simulink model "SNS_WinnerSlice_R8"  (R2025a)
settings: Solver=ode1  StartTime=0.0  StopTime=22  FixedStep=0.002  RelTol=1e-3
libraries: SNS_Library_R2025a x106, simulink x6
(part 1 of 2)
Description:
  | Reduced winner slice: round8_best3.json human circuit in the redesigned SNS_Library architecture. See reports_20261016/sns_simulink/.
settings Model: Creator=ben bolen  LastModifiedBy=ben bolen

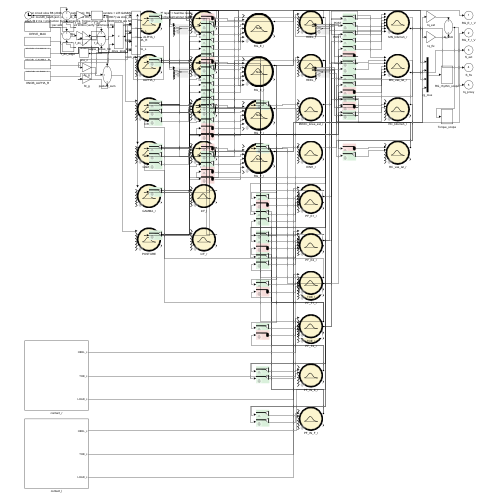
[thumbnail: Simulink's stored preview of the top-level diagram]
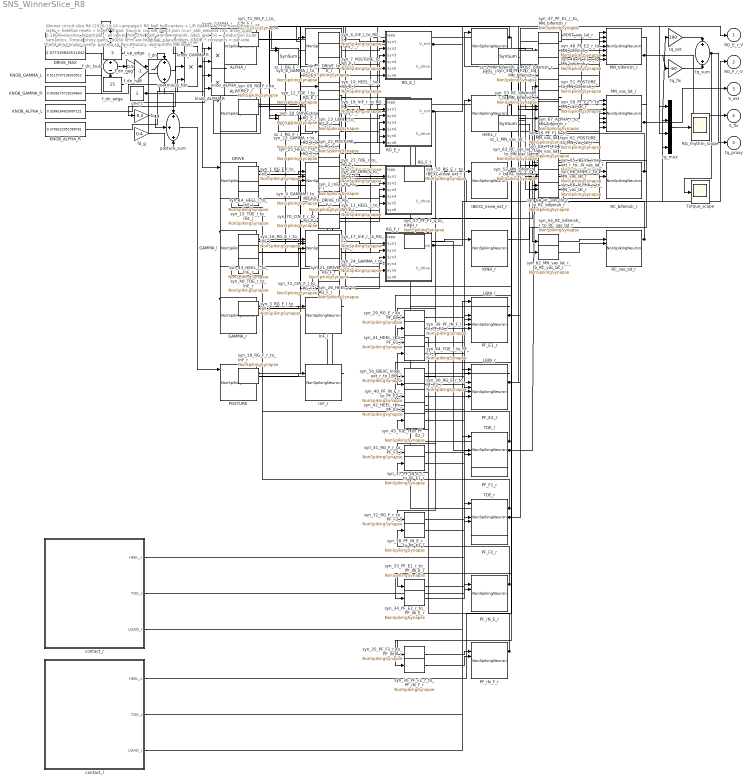
== system SNS_WinnerSlice_R8 ==
  note: Winner circuit slice R8 (2026-10-16 campaign): RG NaP half-centers + L/R GAMMA/ALPHA hand drive + PF layer + heel/toe resets + knee MN pair.
      | Source: round8_best3.json (curr_s8b_wean04 t35, drive_scale 0.3807) via slice_export.json - all values from the built winner network.
      | ode1 @ 2 ms = production Euler semantics. Torque proxy gains 190/60 N*m are NOMINAL placeholders.
      | KNOB_* constants = per-side hand-drive knobs (verify: gamma x4 flips RG duty; alpha shifts MN level).
  ALPHA_l : SNS_Library_R2025a/NonSpikingNeuron  Vrest=0  Gm=1  Cm=100  Thr=0  Slope=5
  ALPHA_r : SNS_Library_R2025a/NonSpikingNeuron  Vrest=0  Gm=1  Cm=100  Thr=0  Slope=5
  CIN_F_l : SNS_Library_R2025a/NonSpikingNeuron  Vrest=0  Gm=1  Cm=50  Thr=0  Slope=5
  CIN_F_r : SNS_Library_R2025a/NonSpikingNeuron  Vrest=0  Gm=1  Cm=50  Thr=0  Slope=5
  DRIVE : SNS_Library_R2025a/NonSpikingNeuron  Vrest=0  Gm=1  Cm=100  Thr=0  Slope=5
  DRIVE_MAX : Constant  Value=2.077319843511042
  GAMMA_l : SNS_Library_R2025a/NonSpikingNeuron  Vrest=0  Gm=1  Cm=100  Thr=0  Slope=5
  GAMMA_r : SNS_Library_R2025a/NonSpikingNeuron  Vrest=0  Gm=1  Cm=100  Thr=0  Slope=5
  HEEL_l : SNS_Library_R2025a/NonSpikingNeuron  Vrest=0  Gm=1  Cm=40  Thr=0  Slope=5
  HEEL_r : SNS_Library_R2025a/NonSpikingNeuron  Vrest=0  Gm=1  Cm=40  Thr=0  Slope=5
  IBEXC_knee_ext_r : SNS_Library_R2025a/NonSpikingNeuron  Vrest=0  Gm=1  Cm=50  Thr=0  Slope=5
  InE_l : SNS_Library_R2025a/NonSpikingNeuron  Vrest=0  Gm=1  Cm=50  Thr=0  Slope=5
  InE_r : SNS_Library_R2025a/NonSpikingNeuron  Vrest=0  Gm=1  Cm=50  Thr=0  Slope=5
  InF_l : SNS_Library_R2025a/NonSpikingNeuron  Vrest=0  Gm=1  Cm=50  Thr=0  Slope=5
  InF_r : SNS_Library_R2025a/NonSpikingNeuron  Vrest=0  Gm=1  Cm=50  Thr=0  Slope=5
  KINH_r : SNS_Library_R2025a/NonSpikingNeuron  Vrest=0  Gm=1  Cm=50  Thr=0  Slope=5
  KNOB_ALPHA_L : Constant  Value=0.3286184629397121
  KNOB_ALPHA_R : Constant  Value=0.3706222051599761
  KNOB_GAMMA_L : Constant  Value=0.5115737136333512
  KNOB_GAMMA_R : Constant  Value=0.3036175720234663
  LBIN_l : SNS_Library_R2025a/NonSpikingNeuron  Vrest=0  Gm=1  Cm=50  Thr=0  Slope=5
  LBIN_r : SNS_Library_R2025a/NonSpikingNeuron  Vrest=0  Gm=1  Cm=50  Thr=0  Slope=5
  MN_bifemsh_r : SNS_Library_R2025a/NonSpikingNeuron  Vrest=0  Gm=1  Cm=30  Thr=0  Slope=5
  MN_vas_lat_r : SNS_Library_R2025a/NonSpikingNeuron  Vrest=0  Gm=1  Cm=30  Thr=0  Slope=5
  PF_E1_r : SNS_Library_R2025a/NonSpikingNeuron  Vrest=0  Gm=1  Cm=48  Thr=0  Slope=5
  PF_E2_r : SNS_Library_R2025a/NonSpikingNeuron  Vrest=0  Gm=1  Cm=72  Thr=0  Slope=5
  PF_F1_r : SNS_Library_R2025a/NonSpikingNeuron  Vrest=0  Gm=1  Cm=72  Thr=0  Slope=5
  PF_F2_r : SNS_Library_R2025a/NonSpikingNeuron  Vrest=0  Gm=1  Cm=128  Thr=0  Slope=5
  PF_IN_E_r : SNS_Library_R2025a/NonSpikingNeuron  Vrest=0  Gm=1  Cm=80  Thr=0  Slope=5
  PF_IN_F_r : SNS_Library_R2025a/NonSpikingNeuron  Vrest=0  Gm=1  Cm=80  Thr=0  Slope=5
  POSTURE : SNS_Library_R2025a/NonSpikingNeuron  Vrest=0  Gm=1  Cm=100  Thr=0  Slope=5
  POST_bifemsh_r : Constant  Value=0
  POST_vas_lat_r : Constant  Value=0
  RC_bifemsh_r : SNS_Library_R2025a/NonSpikingNeuron  Vrest=0  Gm=1  Cm=30  Thr=0  Slope=5
  RC_vas_lat_r : SNS_Library_R2025a/NonSpikingNeuron  Vrest=0  Gm=1  Cm=30  Thr=0  Slope=5
  RG_E_l : Subsystem  mask(SNS NapNeuron (RG soma)){Vrest=0, Gm=1, Cm=50, Thr=0, Slope=5, gIon=12, eIon=8, kM=1, sM=0.8, eM=2, kH=1, sH=-2, eH=3.5, tauH=842.083318953, h0=0.000911051194401}
      mask prompts: Vrest "Resting potential Vrest (mV)"; Gm "Membrane conductance Gm (uS)"; Cm "Membrane capacitance Cm (nF)"; Thr "Saturation threshold Thr (mV)"; Slope "Saturation slope (1/mV)"; gIon "NaP conductance g_ion (uS)"; eIon "NaP reversal e_ion (mV)"; kM "m-gate k_m"; sM "m-gate slope_m (1/mV)"; eM "m-gate midpoint e_m (mV)"; kH "h-gate k_h"; sH "h-gate slope_h (1/mV)"; eH "h-gate midpoint e_h (mV)"; tauH "h-gate time constant tau_h (ms), FIXED"; h0 "initial h"
      mask help: Persistent-Na non-spiking neuron, fixed tau_h (sns_toolbox NonSpikingNeuronWithPersistentSodiumChannel under SNS_NumpyFixedTau = the production RG stepper). Same port conventions as SNS_Library/NonSpikingNeuron: Iapp [nA] + syn1..6, outputs V [mV] and S(V).
      mask Display:
      | t_ = linspace(0, 2*pi, 73);
      | patch(0.95*cos(t_), 0.95*sin(t_), [0 0 0]);
      | patch(0.84*cos(t_), 0.84*sin(t_), [0.99 0.96 0.81]);
      | x_ = linspace(-0.55, 0.55, 61);
      | y_ = -0.20 + 0.40*exp(-((x_+0.08)/0.26).^2);
      | color('black');
      | plot(x_, y_);
      | plot([-0.55 0.55], [-0.20 -0.20]);
      | disp('NaP');
  RG_E_r : Subsystem  mask(SNS NapNeuron (RG soma)){Vrest=0, Gm=1, Cm=50, Thr=0, Slope=5, gIon=12, eIon=8, kM=1, sM=0.8, eM=2, kH=1, sH=-2, eH=3.5, tauH=842.083318953, h0=0.000911051194401}
      mask prompts: Vrest "Resting potential Vrest (mV)"; Gm "Membrane conductance Gm (uS)"; Cm "Membrane capacitance Cm (nF)"; Thr "Saturation threshold Thr (mV)"; Slope "Saturation slope (1/mV)"; gIon "NaP conductance g_ion (uS)"; eIon "NaP reversal e_ion (mV)"; kM "m-gate k_m"; sM "m-gate slope_m (1/mV)"; eM "m-gate midpoint e_m (mV)"; kH "h-gate k_h"; sH "h-gate slope_h (1/mV)"; eH "h-gate midpoint e_h (mV)"; tauH "h-gate time constant tau_h (ms), FIXED"; h0 "initial h"
      mask help: Persistent-Na non-spiking neuron, fixed tau_h (sns_toolbox NonSpikingNeuronWithPersistentSodiumChannel under SNS_NumpyFixedTau = the production RG stepper). Same port conventions as SNS_Library/NonSpikingNeuron: Iapp [nA] + syn1..6, outputs V [mV] and S(V).
      mask Display:
      | t_ = linspace(0, 2*pi, 73);
      | patch(0.95*cos(t_), 0.95*sin(t_), [0 0 0]);
      | patch(0.84*cos(t_), 0.84*sin(t_), [0.99 0.96 0.81]);
      | x_ = linspace(-0.55, 0.55, 61);
      | y_ = -0.20 + 0.40*exp(-((x_+0.08)/0.26).^2);
      | color('black');
      | plot(x_, y_);
      | plot([-0.55 0.55], [-0.20 -0.20]);
      | disp('NaP');
  RG_F_l : Subsystem  mask(SNS NapNeuron (RG soma)){Vrest=0, Gm=1, Cm=50, Thr=0, Slope=5, gIon=12, eIon=8, kM=1, sM=0.8, eM=2, kH=1, sH=-2, eH=3.5, tauH=842.083318953, h0=0.000911051194401}
      mask prompts: Vrest "Resting potential Vrest (mV)"; Gm "Membrane conductance Gm (uS)"; Cm "Membrane capacitance Cm (nF)"; Thr "Saturation threshold Thr (mV)"; Slope "Saturation slope (1/mV)"; gIon "NaP conductance g_ion (uS)"; eIon "NaP reversal e_ion (mV)"; kM "m-gate k_m"; sM "m-gate slope_m (1/mV)"; eM "m-gate midpoint e_m (mV)"; kH "h-gate k_h"; sH "h-gate slope_h (1/mV)"; eH "h-gate midpoint e_h (mV)"; tauH "h-gate time constant tau_h (ms), FIXED"; h0 "initial h"
      mask help: Persistent-Na non-spiking neuron, fixed tau_h (sns_toolbox NonSpikingNeuronWithPersistentSodiumChannel under SNS_NumpyFixedTau = the production RG stepper). Same port conventions as SNS_Library/NonSpikingNeuron: Iapp [nA] + syn1..6, outputs V [mV] and S(V).
      mask Display:
      | t_ = linspace(0, 2*pi, 73);
      | patch(0.95*cos(t_), 0.95*sin(t_), [0 0 0]);
      | patch(0.84*cos(t_), 0.84*sin(t_), [0.99 0.96 0.81]);
      | x_ = linspace(-0.55, 0.55, 61);
      | y_ = -0.20 + 0.40*exp(-((x_+0.08)/0.26).^2);
      | color('black');
      | plot(x_, y_);
      | plot([-0.55 0.55], [-0.20 -0.20]);
      | disp('NaP');
  RG_F_r : Subsystem  mask(SNS NapNeuron (RG soma)){Vrest=0, Gm=1, Cm=50, Thr=0, Slope=5, gIon=12, eIon=8, kM=1, sM=0.8, eM=2, kH=1, sH=-2, eH=3.5, tauH=842.083318953, h0=0.000911051194401}
      mask prompts: Vrest "Resting potential Vrest (mV)"; Gm "Membrane conductance Gm (uS)"; Cm "Membrane capacitance Cm (nF)"; Thr "Saturation threshold Thr (mV)"; Slope "Saturation slope (1/mV)"; gIon "NaP conductance g_ion (uS)"; eIon "NaP reversal e_ion (mV)"; kM "m-gate k_m"; sM "m-gate slope_m (1/mV)"; eM "m-gate midpoint e_m (mV)"; kH "h-gate k_h"; sH "h-gate slope_h (1/mV)"; eH "h-gate midpoint e_h (mV)"; tauH "h-gate time constant tau_h (ms), FIXED"; h0 "initial h"
      mask help: Persistent-Na non-spiking neuron, fixed tau_h (sns_toolbox NonSpikingNeuronWithPersistentSodiumChannel under SNS_NumpyFixedTau = the production RG stepper). Same port conventions as SNS_Library/NonSpikingNeuron: Iapp [nA] + syn1..6, outputs V [mV] and S(V).
      mask Display:
      | t_ = linspace(0, 2*pi, 73);
      | patch(0.95*cos(t_), 0.95*sin(t_), [0 0 0]);
      | patch(0.84*cos(t_), 0.84*sin(t_), [0.99 0.96 0.81]);
      | x_ = linspace(-0.55, 0.55, 61);
      | y_ = -0.20 + 0.40*exp(-((x_+0.08)/0.26).^2);
      | color('black');
      | plot(x_, y_);
      | plot([-0.55 0.55], [-0.20 -0.20]);
      | disp('NaP');
  RG_rhythm_scope : Scope
  TOE_l : SNS_Library_R2025a/NonSpikingNeuron  Vrest=0  Gm=1  Cm=40  Thr=0  Slope=5
  TOE_r : SNS_Library_R2025a/NonSpikingNeuron  Vrest=0  Gm=1  Cm=40  Thr=0  Slope=5
  Torque_scope : Scope
  clock1 : Clock
  contact_l : Subsystem  Description=Foot-contact script (lag 0.50 cycle): stylized stance pattern, production cadence; runner-shaped port currents incl. contact_onset kicks.
  contact_r : Subsystem  Description=Foot-contact script (lag 0.00 cycle): stylized stance pattern, production cadence; runner-shaped port currents incl. contact_onset kicks.
  drive_prod : Product  Inputs=3
  f_dn : Saturate  UpperLimit=1  LowerLimit=0
  f_dn_edge : Constant  Value=15
  f_dn_half : Gain  Gain=0.5
  f_dn_neg : Gain  Gain=-1
  f_dn_tsub : Sum  Inputs=+-
  f_up : Saturate  UpperLimit=1  LowerLimit=0
  f_up_edge : Constant  Value=3
  f_up_half : Gain  Gain=0.5
  f_up_tsub : Sum  Inputs=+-
  fd_g : Gain  Gain=0.4
  fu_g : Gain  Gain=-0.4
  knob_ALPHA_L : Product
  knob_ALPHA_R : Product
  knob_GAMMA_L : Product
  knob_GAMMA_R : Product
  one_c : Constant
  one_minus_fdn : Sum
  posture_sum : Sum  Inputs=+++
  rg_mux : Mux
  ss_1_MN_bifemsh_r : SNS_Library_R2025a/SynSum
  ss_1_MN_vas_lat_r : SNS_Library_R2025a/SynSum
  ss_1_RG_E_l : SNS_Library_R2025a/SynSum
  ss_1_RG_E_r : SNS_Library_R2025a/SynSum
  syn_10_HEEL_l_to_RG_E_l : SNS_Library_R2025a/NonSpikingSynapse  gmax=1.48275698172  Esyn=8  ThrPre=0  SlopePre=5
  syn_11_HEEL_l_to_RG_F_l : SNS_Library_R2025a/NonSpikingSynapse  gmax=1.48275698172  Esyn=-5  ThrPre=0  SlopePre=5
  syn_12_TOE_l_to_RG_E_l : SNS_Library_R2025a/NonSpikingSynapse  gmax=0.360004607905  Esyn=8  ThrPre=0  SlopePre=5
  syn_13_LBIN_l_to_RG_E_l : SNS_Library_R2025a/NonSpikingSynapse  gmax=0.312219190989  Esyn=8  ThrPre=0  SlopePre=5
  syn_14_HEEL_l_to_InE_l : SNS_Library_R2025a/NonSpikingSynapse  gmax=0.139385875967  Esyn=8  ThrPre=0  SlopePre=5
  syn_15_TOE_l_to_InE_l : SNS_Library_R2025a/NonSpikingSynapse  gmax=0.139385875967  Esyn=8  ThrPre=0  SlopePre=5
  syn_16_RG_E_r_to_InE_r : SNS_Library_R2025a/NonSpikingSynapse  gmax=4  Esyn=8  ThrPre=0  SlopePre=5
  syn_17_InE_r_to_RG_F_r : SNS_Library_R2025a/NonSpikingSynapse  gmax=4  Esyn=-5  ThrPre=0  SlopePre=5
  syn_18_RG_F_r_to_InF_r : SNS_Library_R2025a/NonSpikingSynapse  gmax=4  Esyn=8  ThrPre=0  SlopePre=5
  syn_19_InF_r_to_RG_E_r : SNS_Library_R2025a/NonSpikingSynapse  gmax=4  Esyn=-5  ThrPre=0  SlopePre=5
  syn_1_RG_E_l_to_InE_l : SNS_Library_R2025a/NonSpikingSynapse  gmax=4  Esyn=8  ThrPre=0  SlopePre=5
  syn_20_DRIVE_to_RG_E_r : SNS_Library_R2025a/NonSpikingSynapse  gmax=1.69879678682  Esyn=8  ThrPre=0  SlopePre=5
  syn_21_DRIVE_to_RG_F_r : SNS_Library_R2025a/NonSpikingSynapse  gmax=0.996392653075  Esyn=8  ThrPre=0  SlopePre=5
  syn_22_POSTURE_to_RG_E_r : SNS_Library_R2025a/NonSpikingSynapse  gmax=0.8  Esyn=8  ThrPre=0  SlopePre=5
  syn_23_GAMMA_r_to_RG_E_r : SNS_Library_R2025a/NonSpikingSynapse  gmax=1.69879678682  Esyn=8  ThrPre=0  SlopePre=5
  syn_24_GAMMA_r_to_RG_F_r : SNS_Library_R2025a/NonSpikingSynapse  gmax=0.996392653075  Esyn=8  ThrPre=0  SlopePre=5
  syn_25_HEEL_r_to_RG_E_r : SNS_Library_R2025a/NonSpikingSynapse  gmax=1.48275698172  Esyn=8  ThrPre=0  SlopePre=5
  syn_26_HEEL_r_to_RG_F_r : SNS_Library_R2025a/NonSpikingSynapse  gmax=1.48275698172  Esyn=-5  ThrPre=0  SlopePre=5
  syn_27_TOE_r_to_RG_E_r : SNS_Library_R2025a/NonSpikingSynapse  gmax=0.360004607905  Esyn=8  ThrPre=0  SlopePre=5
  syn_28_LBIN_r_to_RG_E_r : SNS_Library_R2025a/NonSpikingSynapse  gmax=0.312219190989  Esyn=8  ThrPre=0  SlopePre=5
  syn_29_RG_E_r_to_PF_E1_r : SNS_Library_R2025a/NonSpikingSynapse  gmax=2.60051473903  Esyn=8  ThrPre=0  SlopePre=5
  syn_2_InE_l_to_RG_F_l : SNS_Library_R2025a/NonSpikingSynapse  gmax=4  Esyn=-5  ThrPre=0  SlopePre=5
  syn_30_RG_E_r_to_PF_E2_r : SNS_Library_R2025a/NonSpikingSynapse  gmax=2.60051473903  Esyn=8  ThrPre=0  SlopePre=5
  syn_31_RG_F_r_to_PF_F1_r : SNS_Library_R2025a/NonSpikingSynapse  gmax=2.60051473903  Esyn=8  ThrPre=0  SlopePre=5
  syn_32_RG_F_r_to_PF_F2_r : SNS_Library_R2025a/NonSpikingSynapse  gmax=2.60051473903  Esyn=8  ThrPre=0  SlopePre=5
  syn_33_PF_E1_r_to_PF_IN_E_r : SNS_Library_R2025a/NonSpikingSynapse  gmax=4  Esyn=8  ThrPre=0  SlopePre=5
  syn_34_PF_E2_r_to_PF_IN_E_r : SNS_Library_R2025a/NonSpikingSynapse  gmax=4  Esyn=8  ThrPre=0  SlopePre=5
  syn_35_PF_F1_r_to_PF_IN_F_r : SNS_Library_R2025a/NonSpikingSynapse  gmax=4  Esyn=8  ThrPre=0  SlopePre=5
  syn_36_PF_F2_r_to_PF_IN_F_r : SNS_Library_R2025a/NonSpikingSynapse  gmax=4  Esyn=8  ThrPre=0  SlopePre=5
  syn_37_PF_IN_E_r_to_PF_F1_r : SNS_Library_R2025a/NonSpikingSynapse  gmax=4  Esyn=-5  ThrPre=0  SlopePre=5
  syn_38_PF_IN_E_r_to_PF_F2_r : SNS_Library_R2025a/NonSpikingSynapse  gmax=4  Esyn=-5  ThrPre=0  SlopePre=5
  syn_39_PF_IN_F_r_to_PF_E1_r : SNS_Library_R2025a/NonSpikingSynapse  gmax=4  Esyn=-5  ThrPre=0  SlopePre=5
  syn_3_RG_F_l_to_InF_l : SNS_Library_R2025a/NonSpikingSynapse  gmax=4  Esyn=8  ThrPre=0  SlopePre=5
  syn_40_PF_IN_F_r_to_PF_E2_r : SNS_Library_R2025a/NonSpikingSynapse  gmax=4  Esyn=-5  ThrPre=0  SlopePre=5
  syn_41_HEEL_r_to_PF_E1_r : SNS_Library_R2025a/NonSpikingSynapse  gmax=0.139385875967  Esyn=8  ThrPre=0  SlopePre=5
  syn_42_HEEL_r_to_PF_E2_r : SNS_Library_R2025a/NonSpikingSynapse  gmax=0.139385875967  Esyn=8  ThrPre=0  SlopePre=5
  syn_43_HEEL_r_to_InE_r : SNS_Library_R2025a/NonSpikingSynapse  gmax=0.139385875967  Esyn=8  ThrPre=0  SlopePre=5
  syn_44_TOE_r_to_PF_E1_r : SNS_Library_R2025a/NonSpikingSynapse  gmax=0.139385875967  Esyn=8  ThrPre=0  SlopePre=5
  syn_45_TOE_r_to_PF_E2_r : SNS_Library_R2025a/NonSpikingSynapse  gmax=0.139385875967  Esyn=8  ThrPre=0  SlopePre=5
  syn_46_TOE_r_to_InE_r : SNS_Library_R2025a/NonSpikingSynapse  gmax=0.139385875967  Esyn=8  ThrPre=0  SlopePre=5
  syn_47_PF_E1_r_to_MN_bifemsh_r : SNS_Library_R2025a/NonSpikingSynapse  gmax=0.0795738000966  Esyn=8  ThrPre=0  SlopePre=5
  syn_48_PF_E2_r_to_MN_bifemsh_r : SNS_Library_R2025a/NonSpikingSynapse  gmax=0.13334321816  Esyn=8  ThrPre=0  SlopePre=5
  syn_49_PF_F1_r_to_MN_bifemsh_r : SNS_Library_R2025a/NonSpikingSynapse  gmax=0.10378112084  Esyn=8  ThrPre=0  SlopePre=5
  syn_4_InF_l_to_RG_E_l : SNS_Library_R2025a/NonSpikingSynapse  gmax=4  Esyn=-5  ThrPre=0  SlopePre=5
  syn_50_PF_F2_r_to_MN_bifemsh_r : SNS_Library_R2025a/NonSpikingSynapse  gmax=0.125256198911  Esyn=8  ThrPre=0  SlopePre=5
  syn_51_POSTURE_to_MN_bifemsh_r : SNS_Library_R2025a/NonSpikingSynapse  gmax=0.0390152379062  Esyn=8  ThrPre=0  SlopePre=5
  syn_52_MN_bifemsh_r_to_RC_bifemsh_r : SNS_Library_R2025a/NonSpikingSynapse  gmax=1  Esyn=8  ThrPre=0  SlopePre=5
  syn_53_RC_bifemsh_r_to_MN_bifemsh_r : SNS_Library_R2025a/NonSpikingSynapse  gmax=0.5  Esyn=-5  ThrPre=0  SlopePre=5
  syn_54_RC_bifemsh_r_to_RC_vas_lat_r : SNS_Library_R2025a/NonSpikingSynapse  gmax=0.5  Esyn=-5  ThrPre=0  SlopePre=5
  syn_55_RG_E_r_to_IBEXC_knee_ext_r : SNS_Library_R2025a/NonSpikingSynapse  gmax=1  Esyn=8  ThrPre=0  SlopePre=5
  syn_56_IBEXC_knee_ext_r_to_LBIN_r : SNS_Library_R2025a/NonSpikingSynapse  gmax=2  Esyn=8  ThrPre=0  SlopePre=5
  syn_57_PF_F1_r_to_KINH_r : SNS_Library_R2025a/NonSpikingSynapse  gmax=1.5  Esyn=8  ThrPre=0  SlopePre=5
  syn_58_PF_E2_r_to_MN_vas_lat_r : SNS_Library_R2025a/NonSpikingSynapse  gmax=0.0261130468897  Esyn=8  ThrPre=0  SlopePre=5
  syn_59_PF_F1_r_to_MN_vas_lat_r : SNS_Library_R2025a/NonSpikingSynapse  gmax=0.00148159131289  Esyn=8  ThrPre=0  SlopePre=5
  syn_5_DRIVE_to_RG_E_l : SNS_Library_R2025a/NonSpikingSynapse  gmax=1.69879678682  Esyn=8  ThrPre=0  SlopePre=5
  syn_60_PF_F2_r_to_MN_vas_lat_r : SNS_Library_R2025a/NonSpikingSynapse  gmax=0.0119761964459  Esyn=8  ThrPre=0  SlopePre=5
  syn_61_POSTURE_to_MN_vas_lat_r : SNS_Library_R2025a/NonSpikingSynapse  gmax=0.00528903407439  Esyn=8  ThrPre=0  SlopePre=5
  syn_62_MN_vas_lat_r_to_RC_vas_lat_r : SNS_Library_R2025a/NonSpikingSynapse  gmax=1  Esyn=8  ThrPre=0  SlopePre=5
  syn_63_RC_vas_lat_r_to_MN_vas_lat_r : SNS_Library_R2025a/NonSpikingSynapse  gmax=0.5  Esyn=-5  ThrPre=0  SlopePre=5
  syn_64_RC_vas_lat_r_to_RC_bifemsh_r : SNS_Library_R2025a/NonSpikingSynapse  gmax=0.5  Esyn=-5  ThrPre=0  SlopePre=5
  syn_65_IBEXC_knee_ext_r_to_MN_vas_lat_r : SNS_Library_R2025a/NonSpikingSynapse  gmax=0.6  Esyn=8  ThrPre=0  SlopePre=5
  syn_66_KINH_r_to_MN_vas_lat_r : SNS_Library_R2025a/NonSpikingSynapse  gmax=0.178469005721  Esyn=-5  ThrPre=0  SlopePre=5
  syn_67_ALPHA_r_to_MN_bifemsh_r : SNS_Library_R2025a/NonSpikingSynapse  gmax=0.87209936962  Esyn=8  ThrPre=0  SlopePre=5
  syn_68_ALPHA_r_to_MN_vas_lat_r : SNS_Library_R2025a/NonSpikingSynapse  gmax=0.87209936962  Esyn=8  ThrPre=0  SlopePre=5
  syn_69_RG_F_r_to_CIN_F_r : SNS_Library_R2025a/NonSpikingSynapse  gmax=0.4  Esyn=8  ThrPre=0  SlopePre=5
  syn_6_DRIVE_to_RG_F_l : SNS_Library_R2025a/NonSpikingSynapse  gmax=0.996392653075  Esyn=8  ThrPre=0  SlopePre=5
  syn_70_CIN_F_r_to_RG_F_l : SNS_Library_R2025a/NonSpikingSynapse  gmax=0.4  Esyn=-5  ThrPre=0  SlopePre=5
  syn_71_RG_F_l_to_CIN_F_l : SNS_Library_R2025a/NonSpikingSynapse  gmax=0.4  Esyn=8  ThrPre=0  SlopePre=5
  syn_72_CIN_F_l_to_RG_F_r : SNS_Library_R2025a/NonSpikingSynapse  gmax=0.4  Esyn=-5  ThrPre=0  SlopePre=5
  syn_7_POSTURE_to_RG_E_l : SNS_Library_R2025a/NonSpikingSynapse  gmax=0.8  Esyn=8  ThrPre=0  SlopePre=5
  syn_8_GAMMA_l_to_RG_E_l : SNS_Library_R2025a/NonSpikingSynapse  gmax=1.69879678682  Esyn=8  ThrPre=0  SlopePre=5
  syn_9_GAMMA_l_to_RG_F_l : SNS_Library_R2025a/NonSpikingSynapse  gmax=0.996392653075  Esyn=8  ThrPre=0  SlopePre=5
  tq_ext : Gain  Gain=190
  tq_flx : Gain  Gain=-60
  tq_sum : Sum
  RG_E_r_V : Outport
  RG_F_r_V : Outport  Port=2
  S_ext : Outport  Port=3
  S_flx : Outport  Port=4
  tq_proxy : Outport  Port=5
  wires:
  f_up_edge/1 -> f_up_tsub/2
  f_up_tsub/1 -> f_up_half/1
  f_up_half/1 -> f_up/1
  f_dn_edge/1 -> f_dn_tsub/2
  f_dn_tsub/1 -> f_dn_half/1
  f_dn_half/1 -> f_dn/1
  clock1/1 -> f_up_tsub/1, f_dn_tsub/1
  f_dn/1 -> f_dn_neg/1, fd_g/1
  f_dn_neg/1 -> one_minus_fdn/1
  one_c/1 -> one_minus_fdn/2, posture_sum/1
  f_up/1 -> drive_prod/1, fu_g/1
  one_minus_fdn/1 -> drive_prod/2
  DRIVE_MAX/1 -> drive_prod/3
  fu_g/1 -> posture_sum/2
  fd_g/1 -> posture_sum/3
  drive_prod/1 -> knob_GAMMA_L/1, knob_GAMMA_R/1, knob_ALPHA_L/1, knob_ALPHA_R/1, DRIVE/1
  KNOB_GAMMA_L/1 -> knob_GAMMA_L/2
  KNOB_GAMMA_R/1 -> knob_GAMMA_R/2
  KNOB_ALPHA_L/1 -> knob_ALPHA_L/2
  KNOB_ALPHA_R/1 -> knob_ALPHA_R/2
  posture_sum/1 -> POSTURE/1
  knob_GAMMA_R/1 -> GAMMA_r/1
  knob_GAMMA_L/1 -> GAMMA_l/1
  knob_ALPHA_R/1 -> ALPHA_r/1
  knob_ALPHA_L/1 -> ALPHA_l/1
  contact_r/1(HEEL_c) -> HEEL_r/1
  contact_r/2(TOE_c) -> TOE_r/1
  contact_r/3(LOAD_c) -> LBIN_r/1
  contact_l/1(HEEL_c) -> HEEL_l/1
  contact_l/2(TOE_c) -> TOE_l/1
  contact_l/3(LOAD_c) -> LBIN_l/1
  POST_vas_lat_r/1 -> MN_vas_lat_r/1
  POST_bifemsh_r/1 -> MN_bifemsh_r/1
  RG_E_l/1(V_mV) -> syn_1_RG_E_l_to_InE_l/1, rg_mux/3
  InE_l/1 -> syn_2_InE_l_to_RG_F_l/1
  RG_F_l/1(V_mV) -> syn_3_RG_F_l_to_InF_l/1, syn_71_RG_F_l_to_CIN_F_l/1, rg_mux/4
  InF_l/1 -> syn_4_InF_l_to_RG_E_l/1
  DRIVE/1 -> syn_5_DRIVE_to_RG_E_l/1, syn_6_DRIVE_to_RG_F_l/1, syn_20_DRIVE_to_RG_E_r/1, syn_21_DRIVE_to_RG_F_r/1
  POSTURE/1 -> syn_7_POSTURE_to_RG_E_l/1, syn_22_POSTURE_to_RG_E_r/1, syn_51_POSTURE_to_MN_bifemsh_r/1, syn_61_POSTURE_to_MN_vas_lat_r/1
  GAMMA_l/1 -> syn_8_GAMMA_l_to_RG_E_l/1, syn_9_GAMMA_l_to_RG_F_l/1
  HEEL_l/1 -> syn_10_HEEL_l_to_RG_E_l/1, syn_11_HEEL_l_to_RG_F_l/1, syn_14_HEEL_l_to_InE_l/1
  TOE_l/1 -> syn_12_TOE_l_to_RG_E_l/1, syn_15_TOE_l_to_InE_l/1
  LBIN_l/1 -> syn_13_LBIN_l_to_RG_E_l/1
  RG_E_r/1(V_mV) -> syn_16_RG_E_r_to_InE_r/1, syn_29_RG_E_r_to_PF_E1_r/1, syn_30_RG_E_r_to_PF_E2_r/1, syn_55_RG_E_r_to_IBEXC_knee_ext_r/1, RG_E_r_V/1, rg_mux/1
  InE_r/1 -> syn_17_InE_r_to_RG_F_r/1
  RG_F_r/1(V_mV) -> syn_18_RG_F_r_to_InF_r/1, syn_31_RG_F_r_to_PF_F1_r/1, syn_32_RG_F_r_to_PF_F2_r/1, syn_69_RG_F_r_to_CIN_F_r/1, RG_F_r_V/1, rg_mux/2
  InF_r/1 -> syn_19_InF_r_to_RG_E_r/1
  GAMMA_r/1 -> syn_23_GAMMA_r_to_RG_E_r/1, syn_24_GAMMA_r_to_RG_F_r/1
  HEEL_r/1 -> syn_25_HEEL_r_to_RG_E_r/1, syn_26_HEEL_r_to_RG_F_r/1, syn_41_HEEL_r_to_PF_E1_r/1, syn_42_HEEL_r_to_PF_E2_r/1, syn_43_HEEL_r_to_InE_r/1
  TOE_r/1 -> syn_27_TOE_r_to_RG_E_r/1, syn_44_TOE_r_to_PF_E1_r/1, syn_45_TOE_r_to_PF_E2_r/1, syn_46_TOE_r_to_InE_r/1
  LBIN_r/1 -> syn_28_LBIN_r_to_RG_E_r/1
  PF_E1_r/1 -> syn_33_PF_E1_r_to_PF_IN_E_r/1, syn_47_PF_E1_r_to_MN_bifemsh_r/1
  PF_E2_r/1 -> syn_34_PF_E2_r_to_PF_IN_E_r/1, syn_48_PF_E2_r_to_MN_bifemsh_r/1, syn_58_PF_E2_r_to_MN_vas_lat_r/1
  PF_F1_r/1 -> syn_35_PF_F1_r_to_PF_IN_F_r/1, syn_49_PF_F1_r_to_MN_bifemsh_r/1, syn_57_PF_F1_r_to_KINH_r/1, syn_59_PF_F1_r_to_MN_vas_lat_r/1
  PF_F2_r/1 -> syn_36_PF_F2_r_to_PF_IN_F_r/1, syn_50_PF_F2_r_to_MN_bifemsh_r/1, syn_60_PF_F2_r_to_MN_vas_lat_r/1
  PF_IN_E_r/1 -> syn_37_PF_IN_E_r_to_PF_F1_r/1, syn_38_PF_IN_E_r_to_PF_F2_r/1
  PF_IN_F_r/1 -> syn_39_PF_IN_F_r_to_PF_E1_r/1, syn_40_PF_IN_F_r_to_PF_E2_r/1
  MN_bifemsh_r/1 -> syn_52_MN_bifemsh_r_to_RC_bifemsh_r/1
  RC_bifemsh_r/1 -> syn_53_RC_bifemsh_r_to_MN_bifemsh_r/1, syn_54_RC_bifemsh_r_to_RC_vas_lat_r/1
  IBEXC_knee_ext_r/1 -> syn_56_IBEXC_knee_ext_r_to_LBIN_r/1, syn_65_IBEXC_knee_ext_r_to_MN_vas_lat_r/1
  MN_vas_lat_r/1 -> syn_62_MN_vas_lat_r_to_RC_vas_lat_r/1
  RC_vas_lat_r/1 -> syn_63_RC_vas_lat_r_to_MN_vas_lat_r/1, syn_64_RC_vas_lat_r_to_RC_bifemsh_r/1
  KINH_r/1 -> syn_66_KINH_r_to_MN_vas_lat_r/1
  ALPHA_r/1 -> syn_67_ALPHA_r_to_MN_bifemsh_r/1, syn_68_ALPHA_r_to_MN_vas_lat_r/1
  CIN_F_r/1 -> syn_70_CIN_F_r_to_RG_F_l/1
  CIN_F_l/1 -> syn_72_CIN_F_l_to_RG_F_r/1
  syn_71_RG_F_l_to_CIN_F_l/1 -> CIN_F_l/2
  syn_69_RG_F_r_to_CIN_F_r/1 -> CIN_F_r/2
  syn_55_RG_E_r_to_IBEXC_knee_ext_r/1 -> IBEXC_knee_ext_r/2
  syn_1_RG_E_l_to_InE_l/1 -> InE_l/2
  syn_14_HEEL_l_to_InE_l/1 -> InE_l/3
  syn_15_TOE_l_to_InE_l/1 -> InE_l/4
  syn_16_RG_E_r_to_InE_r/1 -> InE_r/2
  syn_43_HEEL_r_to_InE_r/1 -> InE_r/3
  syn_46_TOE_r_to_InE_r/1 -> InE_r/4
  syn_3_RG_F_l_to_InF_l/1 -> InF_l/2
  syn_18_RG_F_r_to_InF_r/1 -> InF_r/2
  syn_57_PF_F1_r_to_KINH_r/1 -> KINH_r/2
  syn_56_IBEXC_knee_ext_r_to_LBIN_r/1 -> LBIN_r/2
  syn_47_PF_E1_r_to_MN_bifemsh_r/1 -> MN_bifemsh_r/2
  syn_48_PF_E2_r_to_MN_bifemsh_r/1 -> MN_bifemsh_r/3
  syn_49_PF_F1_r_to_MN_bifemsh_r/1 -> MN_bifemsh_r/4
  syn_50_PF_F2_r_to_MN_bifemsh_r/1 -> MN_bifemsh_r/5
  syn_51_POSTURE_to_MN_bifemsh_r/1 -> MN_bifemsh_r/6
  syn_53_RC_bifemsh_r_to_MN_bifemsh_r/1 -> ss_1_MN_bifemsh_r/1
  syn_67_ALPHA_r_to_MN_bifemsh_r/1 -> ss_1_MN_bifemsh_r/2
  ss_1_MN_bifemsh_r/1 -> MN_bifemsh_r/7
  syn_58_PF_E2_r_to_MN_vas_lat_r/1 -> MN_vas_lat_r/2
  syn_59_PF_F1_r_to_MN_vas_lat_r/1 -> MN_vas_lat_r/3
  syn_60_PF_F2_r_to_MN_vas_lat_r/1 -> MN_vas_lat_r/4
  syn_61_POSTURE_to_MN_vas_lat_r/1 -> MN_vas_lat_r/5
  syn_63_RC_vas_lat_r_to_MN_vas_lat_r/1 -> MN_vas_lat_r/6
  syn_65_IBEXC_knee_ext_r_to_MN_vas_lat_r/1 -> ss_1_MN_vas_lat_r/1
  syn_66_KINH_r_to_MN_vas_lat_r/1 -> ss_1_MN_vas_lat_r/2
  syn_68_ALPHA_r_to_MN_vas_lat_r/1 -> ss_1_MN_vas_lat_r/3
  ss_1_MN_vas_lat_r/1 -> MN_vas_lat_r/7
  syn_29_RG_E_r_to_PF_E1_r/1 -> PF_E1_r/2
  syn_39_PF_IN_F_r_to_PF_E1_r/1 -> PF_E1_r/3
  syn_41_HEEL_r_to_PF_E1_r/1 -> PF_E1_r/4
  syn_44_TOE_r_to_PF_E1_r/1 -> PF_E1_r/5
  syn_30_RG_E_r_to_PF_E2_r/1 -> PF_E2_r/2
  syn_40_PF_IN_F_r_to_PF_E2_r/1 -> PF_E2_r/3
  syn_42_HEEL_r_to_PF_E2_r/1 -> PF_E2_r/4
  syn_45_TOE_r_to_PF_E2_r/1 -> PF_E2_r/5
  syn_31_RG_F_r_to_PF_F1_r/1 -> PF_F1_r/2
  syn_37_PF_IN_E_r_to_PF_F1_r/1 -> PF_F1_r/3
  syn_32_RG_F_r_to_PF_F2_r/1 -> PF_F2_r/2
  syn_38_PF_IN_E_r_to_PF_F2_r/1 -> PF_F2_r/3
  syn_33_PF_E1_r_to_PF_IN_E_r/1 -> PF_IN_E_r/2
  syn_34_PF_E2_r_to_PF_IN_E_r/1 -> PF_IN_E_r/3
  syn_35_PF_F1_r_to_PF_IN_F_r/1 -> PF_IN_F_r/2
  syn_36_PF_F2_r_to_PF_IN_F_r/1 -> PF_IN_F_r/3
  syn_52_MN_bifemsh_r_to_RC_bifemsh_r/1 -> RC_bifemsh_r/2
  syn_64_RC_vas_lat_r_to_RC_bifemsh_r/1 -> RC_bifemsh_r/3
  syn_54_RC_bifemsh_r_to_RC_vas_lat_r/1 -> RC_vas_lat_r/2
  syn_62_MN_vas_lat_r_to_RC_vas_lat_r/1 -> RC_vas_lat_r/3
  syn_4_InF_l_to_RG_E_l/1 -> RG_E_l/2(syn1)
  syn_5_DRIVE_to_RG_E_l/1 -> RG_E_l/3(syn2)
  syn_7_POSTURE_to_RG_E_l/1 -> RG_E_l/4(syn3)
  syn_8_GAMMA_l_to_RG_E_l/1 -> RG_E_l/5(syn4)
  syn_10_HEEL_l_to_RG_E_l/1 -> RG_E_l/6(syn5)
  syn_12_TOE_l_to_RG_E_l/1 -> ss_1_RG_E_l/1
  syn_13_LBIN_l_to_RG_E_l/1 -> ss_1_RG_E_l/2
  ss_1_RG_E_l/1 -> RG_E_l/7(syn6)
  syn_19_InF_r_to_RG_E_r/1 -> RG_E_r/2(syn1)
  syn_20_DRIVE_to_RG_E_r/1 -> RG_E_r/3(syn2)
  syn_22_POSTURE_to_RG_E_r/1 -> RG_E_r/4(syn3)
  syn_23_GAMMA_r_to_RG_E_r/1 -> RG_E_r/5(syn4)
  syn_25_HEEL_r_to_RG_E_r/1 -> RG_E_r/6(syn5)
  syn_27_TOE_r_to_RG_E_r/1 -> ss_1_RG_E_r/1
  syn_28_LBIN_r_to_RG_E_r/1 -> ss_1_RG_E_r/2
  ss_1_RG_E_r/1 -> RG_E_r/7(syn6)
  syn_2_InE_l_to_RG_F_l/1 -> RG_F_l/2(syn1)
  syn_6_DRIVE_to_RG_F_l/1 -> RG_F_l/3(syn2)
  syn_9_GAMMA_l_to_RG_F_l/1 -> RG_F_l/4(syn3)
  syn_11_HEEL_l_to_RG_F_l/1 -> RG_F_l/5(syn4)
  syn_70_CIN_F_r_to_RG_F_l/1 -> RG_F_l/6(syn5)
  syn_17_InE_r_to_RG_F_r/1 -> RG_F_r/2(syn1)
  syn_21_DRIVE_to_RG_F_r/1 -> RG_F_r/3(syn2)
  syn_24_GAMMA_r_to_RG_F_r/1 -> RG_F_r/4(syn3)
  syn_26_HEEL_r_to_RG_F_r/1 -> RG_F_r/5(syn4)
  syn_72_CIN_F_l_to_RG_F_r/1 -> RG_F_r/6(syn5)
  MN_vas_lat_r/2 -> tq_ext/1, S_ext/1
  MN_bifemsh_r/2 -> tq_flx/1, S_flx/1
  tq_ext/1 -> tq_sum/1
  tq_flx/1 -> tq_sum/2
  tq_sum/1 -> tq_proxy/1, Torque_scope/1
  rg_mux/1 -> RG_rhythm_scope/1

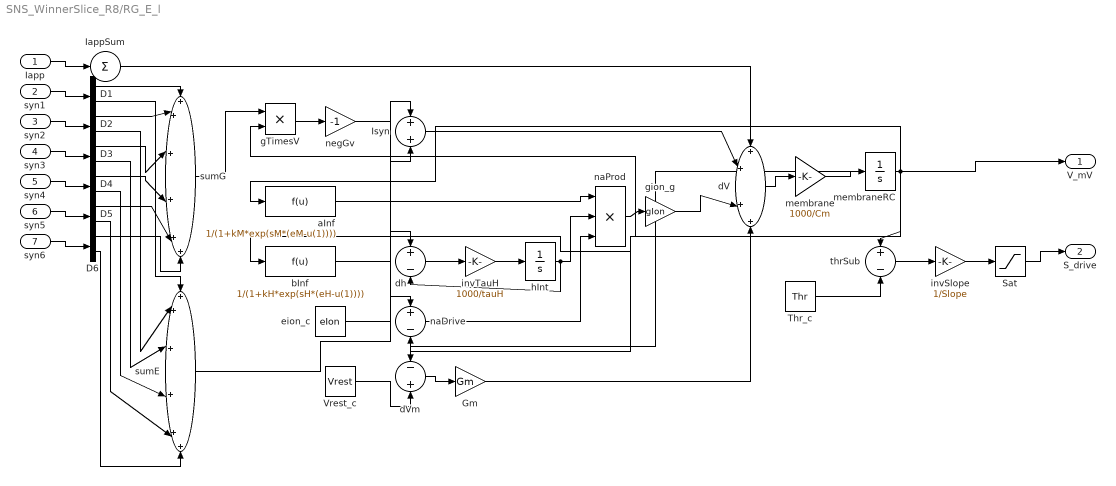
== system SNS_WinnerSlice_R8/RG_E_l ==
  Iapp : Inport
  syn1 : Inport  Port=2  PortDimensions=2
  syn2 : Inport  Port=3  PortDimensions=2
  syn3 : Inport  Port=4  PortDimensions=2
  syn4 : Inport  Port=5  PortDimensions=2
  syn5 : Inport  Port=6  PortDimensions=2
  syn6 : Inport  Port=7  PortDimensions=2
  D{1..6} (6 alike) : Demux  Outputs=2
  Gm : Gain  Gain=Gm
  IappSum : Sum  Inputs=+
  Isyn : Sum
  Sat : Saturate  UpperLimit=1  LowerLimit=0
  Thr_c : Constant  Value=Thr
  Vrest_c : Constant  Value=Vrest
  aInf : Fcn  Expr=1/(1+kM*exp(sM*(eM-u(1))))
  bInf : Fcn  Expr=1/(1+kH*exp(sH*(eH-u(1))))
  dV : Sum  Inputs=++++
  dVm : Sum  Inputs=-+
  dh : Sum  Inputs=+-
  eion_c : Constant  Value=eIon
  gTimesV : Product
  gion_g : Gain  Gain=gIon
  hInt : Integrator  InitialCondition=h0
  invSlope : Gain  Gain=1/Slope
  invTauH : Gain  Gain=1000/tauH
  membrane : Gain  Gain=1000/Cm
  membraneRC : Integrator  InitialCondition=Vrest
  naDrive : Sum  Inputs=+-
  naProd : Product  Inputs=3
  negGv : Gain  Gain=-1
  sumE : Sum  Inputs=++++++
  sumG : Sum  Inputs=++++++
  thrSub : Sum  Inputs=+-
  V_mV : Outport
  S_drive : Outport  Port=2
  wires:
  syn1/1 -> D1/1
  syn2/1 -> D2/1
  syn3/1 -> D3/1
  syn4/1 -> D4/1
  syn5/1 -> D5/1
  syn6/1 -> D6/1
  D1/1 -> sumG/1
  D1/2 -> sumE/1
  D2/1 -> sumG/2
  D2/2 -> sumE/2
  D3/1 -> sumG/3
  D3/2 -> sumE/3
  D4/1 -> sumG/4
  D4/2 -> sumE/4
  D5/1 -> sumG/5
  D5/2 -> sumE/5
  D6/1 -> sumG/6
  D6/2 -> sumE/6
  Iapp/1 -> IappSum/1
  IappSum/1 -> dV/1
  sumG/1 -> gTimesV/1
  membraneRC/1 -> gTimesV/2, aInf/1, bInf/1, naDrive/2, dVm/1, V_mV/1, thrSub/1
  gTimesV/1 -> negGv/1
  sumE/1 -> Isyn/1
  negGv/1 -> Isyn/2
  Isyn/1 -> dV/2
  bInf/1 -> dh/1
  hInt/1 -> dh/2, naProd/2
  dh/1 -> invTauH/1
  invTauH/1 -> hInt/1
  eion_c/1 -> naDrive/1
  aInf/1 -> naProd/1
  naDrive/1 -> naProd/3
  naProd/1 -> gion_g/1
  gion_g/1 -> dV/3
  Vrest_c/1 -> dVm/2
  dVm/1 -> Gm/1
  Gm/1 -> dV/4
  dV/1 -> membrane/1
  membrane/1 -> membraneRC/1
  Thr_c/1 -> thrSub/2
  thrSub/1 -> invSlope/1
  invSlope/1 -> Sat/1
  Sat/1 -> S_drive/1

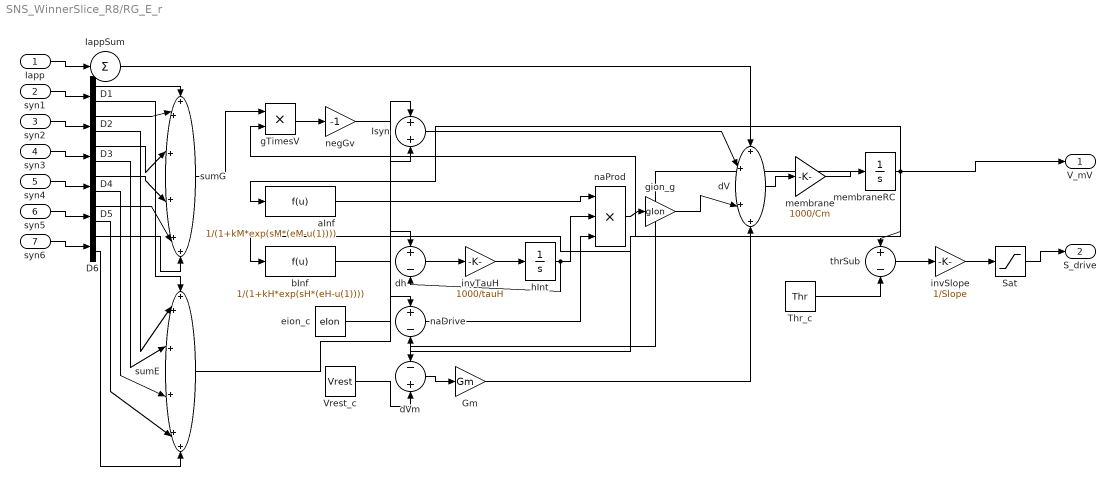
== system SNS_WinnerSlice_R8/RG_E_r ==
  Iapp : Inport
  syn1 : Inport  Port=2  PortDimensions=2
  syn2 : Inport  Port=3  PortDimensions=2
  syn3 : Inport  Port=4  PortDimensions=2
  syn4 : Inport  Port=5  PortDimensions=2
  syn5 : Inport  Port=6  PortDimensions=2
  syn6 : Inport  Port=7  PortDimensions=2
  D{1..6} (6 alike) : Demux  Outputs=2
  Gm : Gain  Gain=Gm
  IappSum : Sum  Inputs=+
  Isyn : Sum
  Sat : Saturate  UpperLimit=1  LowerLimit=0
  Thr_c : Constant  Value=Thr
  Vrest_c : Constant  Value=Vrest
  aInf : Fcn  Expr=1/(1+kM*exp(sM*(eM-u(1))))
  bInf : Fcn  Expr=1/(1+kH*exp(sH*(eH-u(1))))
  dV : Sum  Inputs=++++
  dVm : Sum  Inputs=-+
  dh : Sum  Inputs=+-
  eion_c : Constant  Value=eIon
  gTimesV : Product
  gion_g : Gain  Gain=gIon
  hInt : Integrator  InitialCondition=h0
  invSlope : Gain  Gain=1/Slope
  invTauH : Gain  Gain=1000/tauH
  membrane : Gain  Gain=1000/Cm
  membraneRC : Integrator  InitialCondition=Vrest
  naDrive : Sum  Inputs=+-
  naProd : Product  Inputs=3
  negGv : Gain  Gain=-1
  sumE : Sum  Inputs=++++++
  sumG : Sum  Inputs=++++++
  thrSub : Sum  Inputs=+-
  V_mV : Outport
  S_drive : Outport  Port=2
  wires:
  syn1/1 -> D1/1
  syn2/1 -> D2/1
  syn3/1 -> D3/1
  syn4/1 -> D4/1
  syn5/1 -> D5/1
  syn6/1 -> D6/1
  D1/1 -> sumG/1
  D1/2 -> sumE/1
  D2/1 -> sumG/2
  D2/2 -> sumE/2
  D3/1 -> sumG/3
  D3/2 -> sumE/3
  D4/1 -> sumG/4
  D4/2 -> sumE/4
  D5/1 -> sumG/5
  D5/2 -> sumE/5
  D6/1 -> sumG/6
  D6/2 -> sumE/6
  Iapp/1 -> IappSum/1
  IappSum/1 -> dV/1
  sumG/1 -> gTimesV/1
  membraneRC/1 -> gTimesV/2, aInf/1, bInf/1, naDrive/2, dVm/1, V_mV/1, thrSub/1
  gTimesV/1 -> negGv/1
  sumE/1 -> Isyn/1
  negGv/1 -> Isyn/2
  Isyn/1 -> dV/2
  bInf/1 -> dh/1
  hInt/1 -> dh/2, naProd/2
  dh/1 -> invTauH/1
  invTauH/1 -> hInt/1
  eion_c/1 -> naDrive/1
  aInf/1 -> naProd/1
  naDrive/1 -> naProd/3
  naProd/1 -> gion_g/1
  gion_g/1 -> dV/3
  Vrest_c/1 -> dVm/2
  dVm/1 -> Gm/1
  Gm/1 -> dV/4
  dV/1 -> membrane/1
  membrane/1 -> membraneRC/1
  Thr_c/1 -> thrSub/2
  thrSub/1 -> invSlope/1
  invSlope/1 -> Sat/1
  Sat/1 -> S_drive/1

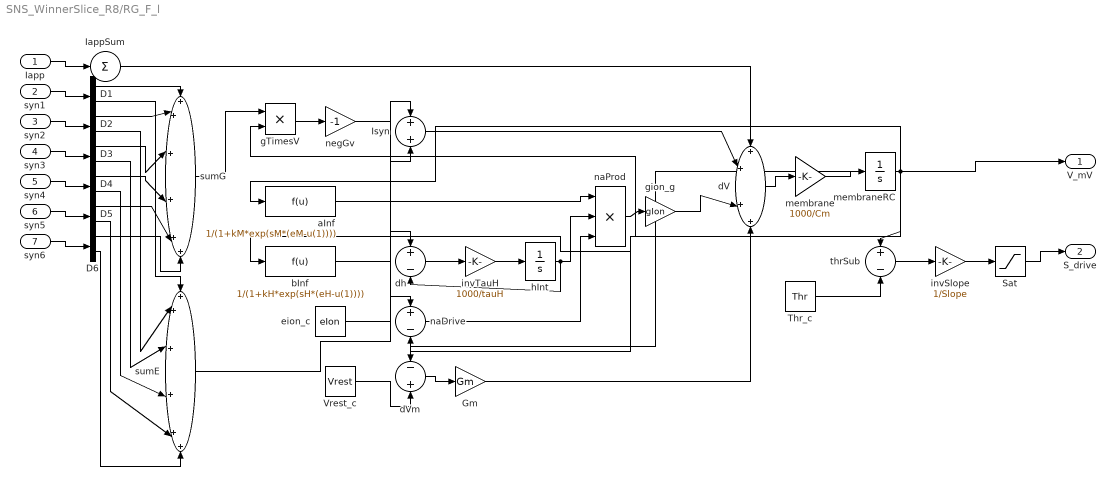
== system SNS_WinnerSlice_R8/RG_F_l ==
  Iapp : Inport
  syn1 : Inport  Port=2  PortDimensions=2
  syn2 : Inport  Port=3  PortDimensions=2
  syn3 : Inport  Port=4  PortDimensions=2
  syn4 : Inport  Port=5  PortDimensions=2
  syn5 : Inport  Port=6  PortDimensions=2
  syn6 : Inport  Port=7  PortDimensions=2
  D{1..6} (6 alike) : Demux  Outputs=2
  Gm : Gain  Gain=Gm
  IappSum : Sum  Inputs=+
  Isyn : Sum
  Sat : Saturate  UpperLimit=1  LowerLimit=0
  Thr_c : Constant  Value=Thr
  Vrest_c : Constant  Value=Vrest
  aInf : Fcn  Expr=1/(1+kM*exp(sM*(eM-u(1))))
  bInf : Fcn  Expr=1/(1+kH*exp(sH*(eH-u(1))))
  dV : Sum  Inputs=++++
  dVm : Sum  Inputs=-+
  dh : Sum  Inputs=+-
  eion_c : Constant  Value=eIon
  gTimesV : Product
  gion_g : Gain  Gain=gIon
  hInt : Integrator  InitialCondition=h0
  invSlope : Gain  Gain=1/Slope
  invTauH : Gain  Gain=1000/tauH
  membrane : Gain  Gain=1000/Cm
  membraneRC : Integrator  InitialCondition=Vrest
  naDrive : Sum  Inputs=+-
  naProd : Product  Inputs=3
  negGv : Gain  Gain=-1
  sumE : Sum  Inputs=++++++
  sumG : Sum  Inputs=++++++
  thrSub : Sum  Inputs=+-
  V_mV : Outport
  S_drive : Outport  Port=2
  wires:
  syn1/1 -> D1/1
  syn2/1 -> D2/1
  syn3/1 -> D3/1
  syn4/1 -> D4/1
  syn5/1 -> D5/1
  syn6/1 -> D6/1
  D1/1 -> sumG/1
  D1/2 -> sumE/1
  D2/1 -> sumG/2
  D2/2 -> sumE/2
  D3/1 -> sumG/3
  D3/2 -> sumE/3
  D4/1 -> sumG/4
  D4/2 -> sumE/4
  D5/1 -> sumG/5
  D5/2 -> sumE/5
  D6/1 -> sumG/6
  D6/2 -> sumE/6
  Iapp/1 -> IappSum/1
  IappSum/1 -> dV/1
  sumG/1 -> gTimesV/1
  membraneRC/1 -> gTimesV/2, aInf/1, bInf/1, naDrive/2, dVm/1, V_mV/1, thrSub/1
  gTimesV/1 -> negGv/1
  sumE/1 -> Isyn/1
  negGv/1 -> Isyn/2
  Isyn/1 -> dV/2
  bInf/1 -> dh/1
  hInt/1 -> dh/2, naProd/2
  dh/1 -> invTauH/1
  invTauH/1 -> hInt/1
  eion_c/1 -> naDrive/1
  aInf/1 -> naProd/1
  naDrive/1 -> naProd/3
  naProd/1 -> gion_g/1
  gion_g/1 -> dV/3
  Vrest_c/1 -> dVm/2
  dVm/1 -> Gm/1
  Gm/1 -> dV/4
  dV/1 -> membrane/1
  membrane/1 -> membraneRC/1
  Thr_c/1 -> thrSub/2
  thrSub/1 -> invSlope/1
  invSlope/1 -> Sat/1
  Sat/1 -> S_drive/1

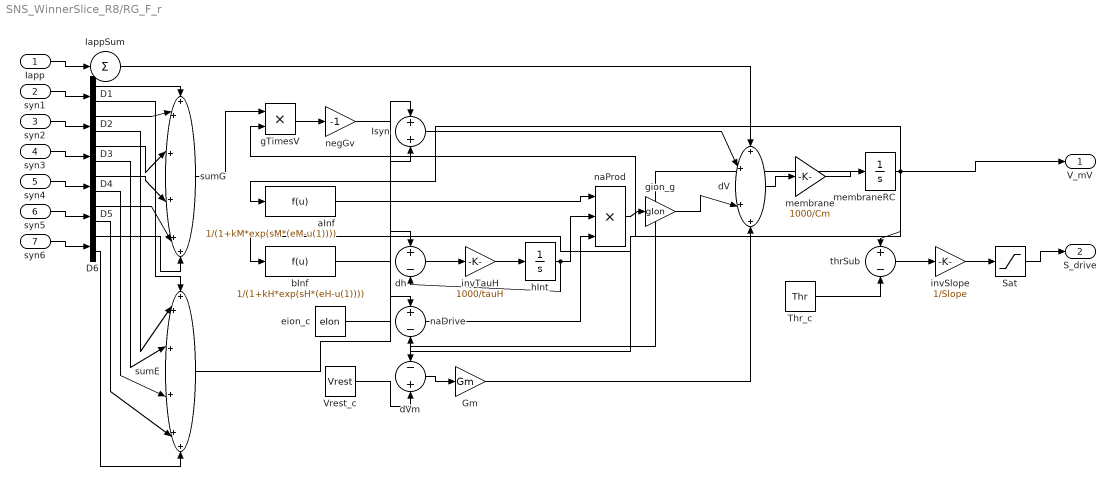
== system SNS_WinnerSlice_R8/RG_F_r ==
  Iapp : Inport
  syn1 : Inport  Port=2  PortDimensions=2
  syn2 : Inport  Port=3  PortDimensions=2
  syn3 : Inport  Port=4  PortDimensions=2
  syn4 : Inport  Port=5  PortDimensions=2
  syn5 : Inport  Port=6  PortDimensions=2
  syn6 : Inport  Port=7  PortDimensions=2
  D{1..6} (6 alike) : Demux  Outputs=2
  Gm : Gain  Gain=Gm
  IappSum : Sum  Inputs=+
  Isyn : Sum
  Sat : Saturate  UpperLimit=1  LowerLimit=0
  Thr_c : Constant  Value=Thr
  Vrest_c : Constant  Value=Vrest
  aInf : Fcn  Expr=1/(1+kM*exp(sM*(eM-u(1))))
  bInf : Fcn  Expr=1/(1+kH*exp(sH*(eH-u(1))))
  dV : Sum  Inputs=++++
  dVm : Sum  Inputs=-+
  dh : Sum  Inputs=+-
  eion_c : Constant  Value=eIon
  gTimesV : Product
  gion_g : Gain  Gain=gIon
  hInt : Integrator  InitialCondition=h0
  invSlope : Gain  Gain=1/Slope
  invTauH : Gain  Gain=1000/tauH
  membrane : Gain  Gain=1000/Cm
  membraneRC : Integrator  InitialCondition=Vrest
  naDrive : Sum  Inputs=+-
  naProd : Product  Inputs=3
  negGv : Gain  Gain=-1
  sumE : Sum  Inputs=++++++
  sumG : Sum  Inputs=++++++
  thrSub : Sum  Inputs=+-
  V_mV : Outport
  S_drive : Outport  Port=2
  wires:
  syn1/1 -> D1/1
  syn2/1 -> D2/1
  syn3/1 -> D3/1
  syn4/1 -> D4/1
  syn5/1 -> D5/1
  syn6/1 -> D6/1
  D1/1 -> sumG/1
  D1/2 -> sumE/1
  D2/1 -> sumG/2
  D2/2 -> sumE/2
  D3/1 -> sumG/3
  D3/2 -> sumE/3
  D4/1 -> sumG/4
  D4/2 -> sumE/4
  D5/1 -> sumG/5
  D5/2 -> sumE/5
  D6/1 -> sumG/6
  D6/2 -> sumE/6
  Iapp/1 -> IappSum/1
  IappSum/1 -> dV/1
  sumG/1 -> gTimesV/1
  membraneRC/1 -> gTimesV/2, aInf/1, bInf/1, naDrive/2, dVm/1, V_mV/1, thrSub/1
  gTimesV/1 -> negGv/1
  sumE/1 -> Isyn/1
  negGv/1 -> Isyn/2
  Isyn/1 -> dV/2
  bInf/1 -> dh/1
  hInt/1 -> dh/2, naProd/2
  dh/1 -> invTauH/1
  invTauH/1 -> hInt/1
  eion_c/1 -> naDrive/1
  aInf/1 -> naProd/1
  naDrive/1 -> naProd/3
  naProd/1 -> gion_g/1
  gion_g/1 -> dV/3
  Vrest_c/1 -> dVm/2
  dVm/1 -> Gm/1
  Gm/1 -> dV/4
  dV/1 -> membrane/1
  membrane/1 -> membraneRC/1
  Thr_c/1 -> thrSub/2
  thrSub/1 -> invSlope/1
  invSlope/1 -> Sat/1
  Sat/1 -> S_drive/1

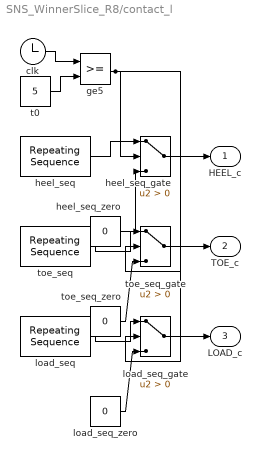
== system SNS_WinnerSlice_R8/contact_l ==
  clk : Clock
  ge5 : RelationalOperator  OutDataTypeStr=boolean  RndMeth=Simplest  InputSameDT=off
  heel_seq : simulink/Sources/Repeating Sequence  rep_seq_t=[0 0.008642 0.017284 0.025926 0.034568 0.04321 0.051852 0.060494 0.069136 0.077778 0.08642 0.095062 0.103704 0.112346 0.120988 0.12963 0.138272 0.146914 0.155556 0.164198 0.17284 0.181482 0.190124 0.198766 0.207408 0.21605 0.224692 0.233334 0.241976 0.250618 0.25926 0.267902 0.276544 0.285186 0.293828 0.30247 0.311112 0.319754 0.328396 0.337038 0.34568 0.354322 0.362964 0.371606 0.380248 0.38889 0.397532 0.406174 0.414816 0.423458 0.4321 0.440742 0.449384 0.458026 0.466668 0.47531 0.483952 0.492594 0.501236 0.509878 0.51852 0.527162 0.535804 0.544446 0.553088 0.56173 0.570372 0.579014 0.587656 0.596298 0.60494 0.613582 0.622224 0.630866 0.639508 0.64815 0.656792 0.665434 0.674076 0.682718 0.69136 0.700002 0.708644 0.717286 0.725928 0.73457 0.743212 0.751854 0.760496 0.769138 0.77778 0.786422 0.795064 0.803706 0.812348 0.82099 0.829632 0.838274 0.846916 0.855558 0.8642 0.872842 0.881484 0.890126 0.898768 0.90741 0.916052 0.924694 0.933336 0.941978 0.95062 0.959262 0.967904 0.976546 0.985188 0.99383 1.002472 1.011114 1.019756 1.028398 1.03704 1.045682 1.054324 1.062966 1.071608 1.08025 1.088892 1.097534 1.106176 1.114818 1.12346 1.132102 1.140744 1.149386 1.158028 1.16667 1.175312 1.183954 1.192596 1.201238 1.20988 1.218522 1.227164 1.235806 1.244448 1.25309 1.261732 1.270374 1.279016 1.287658 1.2963 1.304942 1.313584 1.322226 1.330868 1.33951 1.348152 1.356794 1.365436 1.374078 1.38272 1.391362 1.400004 1.408646 1.417288 1.42593 1.434572 1.443214 1.451856 1.460498 1.46914 1.477782 1.486424 1.495066 1.503708 1.51235 1.520992 1.529634 1.538276 1.546918 1.55556 1.564202 1.572844 1.581486 1.590128 1.59877 1.607412 1.616054 1.624696 1.633338 1.64198 1.650622 1.659264 1.667906 1.676548 1.68519 1.693832 1.702474 1.711116 1.719758 1.7284]  rep_seq_y=[0.817272721 1.460274974 2.104220735 2.749077948 2.935867053 2.911684299 2.88832321 2.86575587 2.843955308 2.822895471 2.802551192 2.782898157 2.763912881 2.745572674 2.727855618 2.710740541 2.69420699 2.678235204 2.662806098 2.647901231 2.633502793 2.619593576 2.606156956 2.593176878 2.580637828 2.568524822 2.556823384 2.54551953 2.53459975 2.524050996 2.513860661 2.504016566 2.494506948 2.485320441 2.476446067 2.467873221 2.459591658 2.45159148 2.443863127 2.436397364 2.429185267 2.422218218 2.41548789 2.408986242 2.402705502 2.361334428 2.308401593 2.255667905 2.203126599 2.150771137 2.098595205 2.046592703 1.994757738 1.943084618 1.891567844 1.840202104 1.788982265 1.73790337 1.686960632 1.636149422 1.585465273 1.552320378 1.519294055 1.486382276 1.453581149 1.420886915 1.38829594 1.355804718 1.323409858 1.291108087 1.258896241 1.226771266 1.194730209 1.162770219 1.130888541 1.099082516 1.067349572 1.035687226 1.00409308 0.972564816 0.941100196 0.909697057 0.878353311 0.847066939 0.815835992 0.784658587 0.753532904 0.722457186 0.691429736 0.660448914 0.629513134 0.598620868 0.567770635 0.536961009 0.506190609 0.475458103 0.444762203 0.414101665 0.383475288 0.352881911 0.322320413 0.29178971 0.261288757 0.230816542 0.200372089 0.169954455 0.139562729 0.10919603 0.078853508 0.048534341 0.018237736 0.017618066 0.017019451 0.016441175 0.015882547 0.0153429 0.014821589 0.014317991 0.013831503 0.013361546 0.012907556 0.012468991 0.012045328 0.011636059 0.011240697 0.010858768 0.010489816 0.010133399 0.009789093 0.009456486 0.00913518 0.00882479 0.008524947 0.008235292 0.007955479 0.007685173 0.007424051 0.007171801 0.006928122 0.006692723 0.006465322 0.006245648 0.006033437 0.005828437 -0.817272721 -0.789503958 -0.762678704 -0.736764901 -0.711731581 -0.687548826 -0.664187738 -0.641620397 -0.619819835 -0.598759998 -0.578415719 -0.558762684 -0.539777408 -0.521437201 -0.503720146 -0.486605069 -0.470071517 -0.454099732 -0.438670625 -0.423765759 -0.409367321 -0.395458103 -0.382021484 -0.369041405 -0.356502356 -0.344389349 -0.332687911 -0.321384057 -0.310464278 -0.299915524 -0.289725188 -0.279881094 -0.270371475 -0.261184968 -0.252310595 -0.243737749 -0.235456185 -0.227456008 -0.219727655 -0.212261891 -0.205049794 -0.198082745 -0.191352418 -0.184850769 -0.17857003 -0.172502693 -0.166641508 -0.160979471 -0.155509815 -0.150226003 -0.145121721 -0.140190869 -0.135427555 -0.130826085 -0.126380961 -0.122086871 -0.117938682]
  heel_seq_gate : Switch  Criteria=u2 > Threshold  SaturateOnIntegerOverflow=off  InputSameDT=off
  heel_seq_zero : Constant  Value=0
  load_seq : simulink/Sources/Repeating Sequence  rep_seq_t=[0 0.008642 0.017284 0.025926 0.034568 0.04321 0.051852 0.060494 0.069136 0.077778 0.08642 0.095062 0.103704 0.112346 0.120988 0.12963 0.138272 0.146914 0.155556 0.164198 0.17284 0.181482 0.190124 0.198766 0.207408 0.21605 0.224692 0.233334 0.241976 0.250618 0.25926 0.267902 0.276544 0.285186 0.293828 0.30247 0.311112 0.319754 0.328396 0.337038 0.34568 0.354322 0.362964 0.371606 0.380248 0.38889 0.397532 0.406174 0.414816 0.423458 0.4321 0.440742 0.449384 0.458026 0.466668 0.47531 0.483952 0.492594 0.501236 0.509878 0.51852 0.527162 0.535804 0.544446 0.553088 0.56173 0.570372 0.579014 0.587656 0.596298 0.60494 0.613582 0.622224 0.630866 0.639508 0.64815 0.656792 0.665434 0.674076 0.682718 0.69136 0.700002 0.708644 0.717286 0.725928 0.73457 0.743212 0.751854 0.760496 0.769138 0.77778 0.786422 0.795064 0.803706 0.812348 0.82099 0.829632 0.838274 0.846916 0.855558 0.8642 0.872842 0.881484 0.890126 0.898768 0.90741 0.916052 0.924694 0.933336 0.941978 0.95062 0.959262 0.967904 0.976546 0.985188 0.99383 1.002472 1.011114 1.019756 1.028398 1.03704 1.045682 1.054324 1.062966 1.071608 1.08025 1.088892 1.097534 1.106176 1.114818 1.12346 1.132102 1.140744 1.149386 1.158028 1.16667 1.175312 1.183954 1.192596 1.201238 1.20988 1.218522 1.227164 1.235806 1.244448 1.25309 1.261732 1.270374 1.279016 1.287658 1.2963 1.304942 1.313584 1.322226 1.330868 1.33951 1.348152 1.356794 1.365436 1.374078 1.38272 1.391362 1.400004 1.408646 1.417288 1.42593 1.434572 1.443214 1.451856 1.460498 1.46914 1.477782 1.486424 1.495066 1.503708 1.51235 1.520992 1.529634 1.538276 1.546918 1.55556 1.564202 1.572844 1.581486 1.590128 1.59877 1.607412 1.616054 1.624696 1.633338 1.64198 1.650622 1.659264 1.667906 1.676548 1.68519 1.693832 1.702474 1.711116 1.719758 1.7284]  rep_seq_y=[0 0.082391175 0.164782351 0.247173526 0.329564702 0.411955877 0.468328786 0.468328786 0.468328786 0.468328786 0.468328786 0.465437868 0.459656031 0.453874194 0.448092357 0.442310521 0.436528684 0.430746847 0.42496501 0.419183173 0.413401336 0.407619499 0.401837662 0.396055826 0.390273989 0.384492152 0.378710315 0.372928478 0.367146641 0.361364804 0.355582968 0.349801131 0.344019294 0.338237457 0.33245562 0.326673783 0.320891946 0.315110109 0.309328273 0.303546436 0.297764599 0.291982762 0.286200925 0.280419088 0.274637251 0.268855414 0.263073578 0.257291741 0.251509904 0.245728067 0.23994623 0.234164393 0.228382556 0.22260072 0.216818883 0.211037046 0.205255209 0.199473372 0.193691535 0.187909698 0.182127861 0.184209323 0.186290784 0.188372245 0.190453707 0.192535168 0.194616629 0.19669809 0.198779552 0.200861013 0.202942474 0.205023935 0.207105397 0.209186858 0.211268319 0.213349781 0.215431242 0.217512703 0.219594164 0.221675626 0.223757087 0.225838548 0.227920009 0.230001471 0.232082932 0.234164393 0.236245855 0.238327316 0.240408777 0.242490238 0.2445717 0.246653161 0.248734622 0.250816083 0.252897545 0.254979006 0.257060467 0.259141929 0.26122339 0.263304851 0.265386312 0.267467774 0.269549235 0.271630696 0.273712157 0.275793619 0.27787508 0.279956541 0.282038003 0.284119464 0.286200925 0.286200925 0.286200925 0.286200925 0.286200925 0.286200925 0.286200925 0.286200925 0.286200925 0.286200925 0.286200925 0.286200925 0.286200925 0.286200925 0.286200925 0.299210058 0.312219191 0.325228324 0.338237457 0.35124659 0.364255723 0.377264856 0.390273989 0.403283122 0.416292255 0.429301388 0.442310521 0.455319654 0.468328786 0.468328786 0.468328786 0.370760289 0.247173526 0.123586763 0 0 0 0 0 0 0 0 0 0 0 0 0 0 0 0 0 0 0 0 0 0 0 0 0 0 0 0 0 0 0 0 0 0 0 0 0 0 0 0 0 0 0 0 0 0 0 0 0 0 0 0 0 0 0 0 0]
  load_seq_gate : Switch  Criteria=u2 > Threshold  SaturateOnIntegerOverflow=off  InputSameDT=off
  load_seq_zero : Constant  Value=0
  t0 : Constant  Value=5
  toe_seq : simulink/Sources/Repeating Sequence  rep_seq_t=[0 0.008642 0.017284 0.025926 0.034568 0.04321 0.051852 0.060494 0.069136 0.077778 0.08642 0.095062 0.103704 0.112346 0.120988 0.12963 0.138272 0.146914 0.155556 0.164198 0.17284 0.181482 0.190124 0.198766 0.207408 0.21605 0.224692 0.233334 0.241976 0.250618 0.25926 0.267902 0.276544 0.285186 0.293828 0.30247 0.311112 0.319754 0.328396 0.337038 0.34568 0.354322 0.362964 0.371606 0.380248 0.38889 0.397532 0.406174 0.414816 0.423458 0.4321 0.440742 0.449384 0.458026 0.466668 0.47531 0.483952 0.492594 0.501236 0.509878 0.51852 0.527162 0.535804 0.544446 0.553088 0.56173 0.570372 0.579014 0.587656 0.596298 0.60494 0.613582 0.622224 0.630866 0.639508 0.64815 0.656792 0.665434 0.674076 0.682718 0.69136 0.700002 0.708644 0.717286 0.725928 0.73457 0.743212 0.751854 0.760496 0.769138 0.77778 0.786422 0.795064 0.803706 0.812348 0.82099 0.829632 0.838274 0.846916 0.855558 0.8642 0.872842 0.881484 0.890126 0.898768 0.90741 0.916052 0.924694 0.933336 0.941978 0.95062 0.959262 0.967904 0.976546 0.985188 0.99383 1.002472 1.011114 1.019756 1.028398 1.03704 1.045682 1.054324 1.062966 1.071608 1.08025 1.088892 1.097534 1.106176 1.114818 1.12346 1.132102 1.140744 1.149386 1.158028 1.16667 1.175312 1.183954 1.192596 1.201238 1.20988 1.218522 1.227164 1.235806 1.244448 1.25309 1.261732 1.270374 1.279016 1.287658 1.2963 1.304942 1.313584 1.322226 1.330868 1.33951 1.348152 1.356794 1.365436 1.374078 1.38272 1.391362 1.400004 1.408646 1.417288 1.42593 1.434572 1.443214 1.451856 1.460498 1.46914 1.477782 1.486424 1.495066 1.503708 1.51235 1.520992 1.529634 1.538276 1.546918 1.55556 1.564202 1.572844 1.581486 1.590128 1.59877 1.607412 1.616054 1.624696 1.633338 1.64198 1.650622 1.659264 1.667906 1.676548 1.68519 1.693832 1.702474 1.711116 1.719758 1.7284]  rep_seq_y=[0.817272721 0.789503958 0.762678704 0.736764901 0.711731581 0.687548826 0.664187738 0.641620397 0.619819835 0.598759998 0.578415719 0.558762684 0.539777408 0.521437201 0.503720146 0.486605069 0.470071517 0.454099732 0.438670625 0.423765759 0.409367321 0.395458103 0.382021484 0.369041405 0.356502356 0.344389349 0.332687911 0.321384057 0.310464278 0.299915524 0.289725188 0.279881094 0.270371475 0.261184968 0.252310595 0.243737749 0.235456185 0.227456008 0.219727655 0.212261891 0.205049794 0.198082745 0.191352418 0.184850769 0.17857003 0.172502693 0.166641508 0.160979471 0.155509815 0.150226003 0.145121721 0.140190869 0.135427555 0.130826085 0.126380961 0.122086871 0.117938682 0.113931438 0.110060349 0.10632079 0.102708291 0.107138637 0.111687555 0.116351017 0.121125131 0.126006138 0.130990405 0.136074423 0.141254805 0.146528274 0.15189167 0.157341935 0.162876119 0.16849137 0.174184934 0.179954149 0.185796446 0.191709341 0.197690436 0.203737413 0.209848034 0.216020137 0.222251631 0.2285405 0.234884794 0.24128263 0.247732188 0.254231712 0.260779503 0.267373921 0.274013383 0.280696357 0.287421366 0.294186981 0.300991822 0.307834557 0.314713897 0.321628601 0.328577464 0.335559328 0.342573071 0.34961761 0.356691897 0.363794924 0.370925712 0.378083319 0.385266834 0.392475375 0.399708094 0.406964168 0.414242805 0.413623135 0.413024519 0.412446243 0.411887616 0.411347969 0.410826658 0.41032306 0.409836572 0.409366614 0.408912624 0.40847406 0.408050396 0.407641128 0.407245766 0.424864067 0.442495345 0.460139159 0.477795084 0.495462707 0.513141631 0.530831472 0.548531859 0.548242204 0.547962391 0.547692085 0.547430963 0.547178713 0.546935034 0.546699635 0.546472234 0.519252214 0.348037815 0.176830626 -0.817272721 -0.789503958 -0.762678704 -0.736764901 -0.711731581 -0.687548826 -0.664187738 -0.641620397 -0.619819835 -0.598759998 -0.578415719 -0.558762684 -0.539777408 -0.521437201 -0.503720146 -0.486605069 -0.470071517 -0.454099732 -0.438670625 -0.423765759 -0.409367321 -0.395458103 -0.382021484 -0.369041405 -0.356502356 -0.344389349 -0.332687911 -0.321384057 -0.310464278 -0.299915524 -0.289725188 -0.279881094 -0.270371475 -0.261184968 -0.252310595 -0.243737749 -0.235456185 -0.227456008 -0.219727655 -0.212261891 -0.205049794 -0.198082745 -0.191352418 -0.184850769 -0.17857003 -0.172502693 -0.166641508 -0.160979471 -0.155509815 -0.150226003 -0.145121721 -0.140190869 -0.135427555 -0.130826085 -0.126380961 -0.122086871 -0.117938682]
  toe_seq_gate : Switch  Criteria=u2 > Threshold  SaturateOnIntegerOverflow=off  InputSameDT=off
  toe_seq_zero : Constant  Value=0
  HEEL_c : Outport
  TOE_c : Outport  Port=2
  LOAD_c : Outport  Port=3
  wires:
  clk/1 -> ge5/1
  t0/1 -> ge5/2
  heel_seq/1 -> heel_seq_gate/1
  ge5/1 -> heel_seq_gate/2, toe_seq_gate/2, load_seq_gate/2
  heel_seq_zero/1 -> heel_seq_gate/3
  heel_seq_gate/1 -> HEEL_c/1
  toe_seq/1 -> toe_seq_gate/1
  toe_seq_zero/1 -> toe_seq_gate/3
  toe_seq_gate/1 -> TOE_c/1
  load_seq/1 -> load_seq_gate/1
  load_seq_zero/1 -> load_seq_gate/3
  load_seq_gate/1 -> LOAD_c/1
